simulink model "sr_hysteretic_comparator"  (R2025b)
settings: Solver=ode45  StartTime=0.0  StopTime=0.06  MaxStep=1e-4  RelTol=1e-3
values from neighbouring files (symbols this model uses):
  Vcmd = 2    [latched_hysteretic_circuit_A01.m]
  Vhys = 0.01    [buck_converter_parameters_A01.m]    (also in hysteretic_controller_simu_A01.m = 0.2; latched_hysteretic_circuit_A01.m = 0.5)
settings Model: Creator=arif  LastModifiedBy=arif

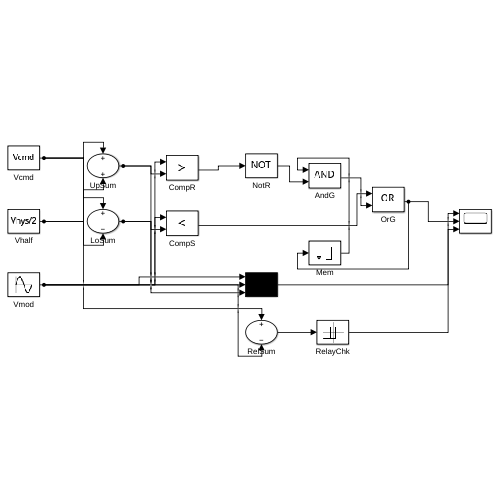
[thumbnail: Simulink's stored preview of the top-level diagram]
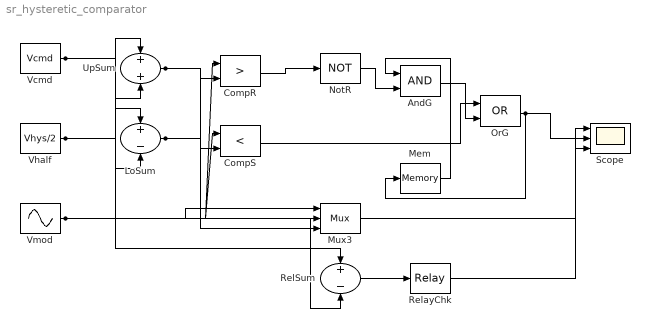
== system sr_hysteretic_comparator ==
  AndG : Logic  AllPortsSameDT=off  OutDataTypeStr=boolean
  CompR : RelationalOperator  Operator=>  OutDataTypeStr=boolean  RndMeth=Simplest  InputSameDT=off
  CompS : RelationalOperator  Operator=<  OutDataTypeStr=boolean  RndMeth=Simplest  InputSameDT=off
  LoSum : Sum  Inputs=+-
  Mem : Memory
  Mux3 : Mux  Inputs=3
  NotR : Logic  Operator=NOT  AllPortsSameDT=off  OutDataTypeStr=boolean
  OrG : Logic  Operator=OR  AllPortsSameDT=off  OutDataTypeStr=boolean
  RelSum : Sum  Inputs=+-
  RelayChk : Relay  OnSwitchValue=Vhys/2  OffSwitchValue=-Vhys/2
  Scope : Scope  NumInputPorts=3
  UpSum : Sum
  Vcmd : Constant  Value=Vcmd
  Vhalf : Constant  Value=Vhys/2
  Vmod : Sin  Bias=Vcmd  Frequency=2*pi*50  SampleTime=0
  wires:
  Vcmd/1 -> UpSum/1, LoSum/1, RelSum/1
  Vhalf/1 -> UpSum/2, LoSum/2
  Vmod/1 -> CompR/1, CompS/1, RelSum/2, Mux3/1
  UpSum/1 -> CompR/2, Mux3/2
  LoSum/1 -> CompS/2, Mux3/3
  CompR/1 -> NotR/1
  NotR/1 -> AndG/2
  Mem/1 -> AndG/1
  AndG/1 -> OrG/2
  CompS/1 -> OrG/1
  OrG/1 -> Mem/1, Scope/2
  RelSum/1 -> RelayChk/1
  Mux3/1 -> Scope/1
  RelayChk/1 -> Scope/3
